simulink model "research_paper_cmrcc"  (R2024b)
settings: Solver=VariableStepAuto  StartTime=0.0  StopTime=0.05  RelTol=1e-3
libraries: spsSeriesRLCBranchLib x9, spsDiodeLib x6, spsCurrentMeasurementLib x5, spsVoltageMeasurementLib x4, spsDCVoltageSourceLib x1, spsGroundLib x1, spsMosfetLib x1, spsMultimeterLib x1, spsMutualInductanceLib x1, eePwmGenerator x1, sps_lib x1
settings Model: Creator=manas  LastModifiedBy=manas

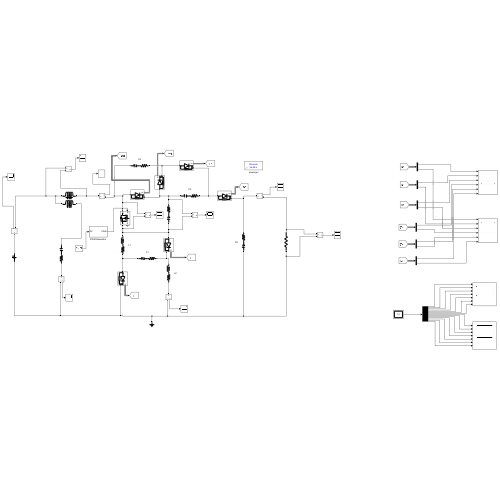
[thumbnail: Simulink's stored preview of the top-level diagram]
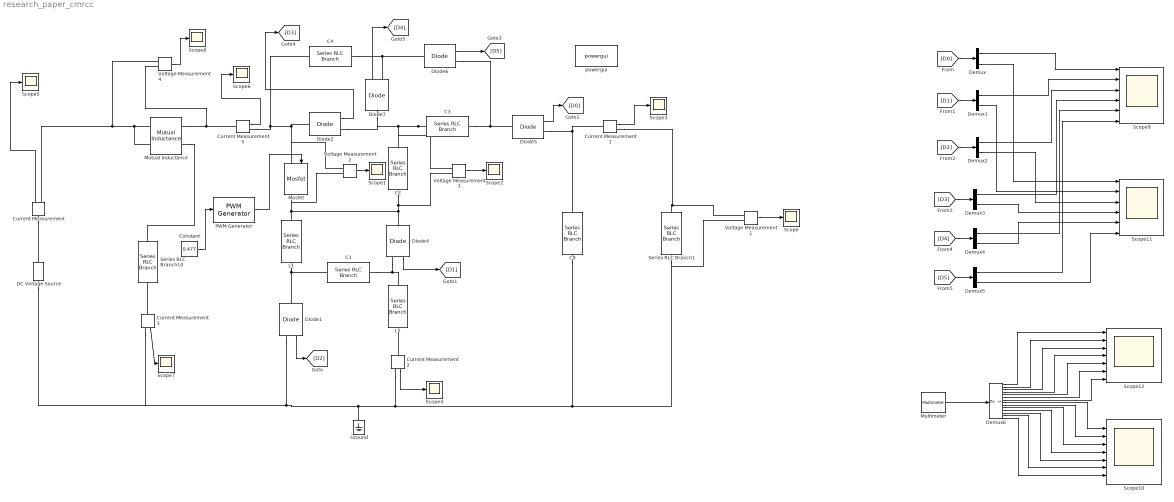
== system research_paper_cmrcc ==
  C0 : spsSeriesRLCBranchLib/Series RLC Branch  LConnTagsString=__new0  RConnTagsString=__new0  BranchType=RC  Resistance=0.05  Inductance=1e-3  SetiL0=off  InitialCurrent=0  Capacitance=100e-6  Setx0=on  InitialVoltage=400  Measurements=Branch voltage and current
  C1 : spsSeriesRLCBranchLib/Series RLC Branch  LConnTagsString=__new0  RConnTagsString=__new0  BranchType=RC  Resistance=0.003  Inductance=1e-3  SetiL0=off  InitialCurrent=0  Capacitance=100e-6  Setx0=on  InitialVoltage=48  Measurements=Branch voltage and current
  C2 : spsSeriesRLCBranchLib/Series RLC Branch  LConnTagsString=__new0  RConnTagsString=__new0  BranchType=RC  Resistance=0.003  Inductance=1e-3  SetiL0=off  InitialCurrent=0  Capacitance=100e-6  Setx0=on  InitialVoltage=176  Measurements=Branch voltage and current
  C3 : spsSeriesRLCBranchLib/Series RLC Branch  LConnTagsString=__new0  RConnTagsString=__new0  BranchType=RC  Resistance=0.003  Inductance=1e-3  SetiL0=off  InitialCurrent=0  Capacitance=100e-6  Setx0=on  InitialVoltage=176  Measurements=Branch voltage and current
  C4 : spsSeriesRLCBranchLib/Series RLC Branch  LConnTagsString=__new0  RConnTagsString=__new0  BranchType=RC  Resistance=0.003  Inductance=1e-3  SetiL0=off  InitialCurrent=0  Capacitance=100e-6  Setx0=on  InitialVoltage=176  Measurements=Branch voltage and current
  Constant : Constant  Value=0.477
  Current Measurement{,1..3,5} (5 alike) : spsCurrentMeasurementLib/Current Measurement  PhasorSimulation=off  OutputType=Complex  PSBequivalent=0
  DC Voltage Source : spsDCVoltageSourceLib/DC Voltage Source  Amplitude=48  Measurements=None
  Demux{,1..5} (6 alike) : Demux  Outputs=2
  Demux6 : Demux  Outputs=14
  Diode1 : spsDiodeLib/Diode  Ron=0.01  Lon=0  Vf=0.85  IC=0  UseSnubber=0  Rs=500  Cs=250e-9  Measurements=on
  Diode{2,5..7} (4 alike) : spsDiodeLib/Diode  Ron=0.01  Lon=0  Vf=0.12  IC=0  UseSnubber=0  Rs=500  Cs=250e-9  Measurements=on
  Diode4 : spsDiodeLib/Diode  Ron=0.01  Lon=0  Vf=0.85  IC=0  UseSnubber=0  Rs=500  Cs=250e-9  Measurements=on
  Ground : spsGroundLib/Ground  LConnTagsString=a
  L1 : spsSeriesRLCBranchLib/Series RLC Branch  LConnTagsString=__new0  RConnTagsString=__new0  BranchType=RL  Resistance=0.12  Inductance=750e-6  SetiL0=on  InitialCurrent=-2.57  Capacitance=1e-6  Setx0=off  InitialVoltage=0  Measurements=Branch voltage and current
  L2 : spsSeriesRLCBranchLib/Series RLC Branch  LConnTagsString=__new0  RConnTagsString=__new0  BranchType=RL  Resistance=0.12  Inductance=750e-6  SetiL0=on  InitialCurrent=-2.57  Capacitance=1e-6  Setx0=off  InitialVoltage=0  Measurements=Branch voltage and current
  Mosfet : spsMosfetLib/Mosfet  Ron=0.016  Lon=0  Rd=0.01  Vfd=0  IC=0  Rs=1e5  Cs=inf  Measurements=on
  Multimeter : spsMultimeterLib/Multimeter  L=14  sel=[1 2 3 4 5 6 7 8 9 10 11 12 13 14]  yselected={}  Gain=[1 1 1 1 1 1 1 1 1 1 1 1 1 1]  OutputType=Complex  PlotAtSimulationStop=off  PhasorSimulation=off
  Mutual Inductance : spsMutualInductanceLib/Mutual Inductance  LConnTagsString=a|b  RConnTagsString=A|B  TypeOfMutual=Two or three windings with equal mutual terms  NumberOfWindings=3  SelfImpedance1=[0.014 1.5e-6]  SelfImpedance2=[0.014 1.5e-6]  ThreeWindings=off  SelfImpedance3=[ 1.1 1.1e-03]  MutualImpedance=[0 1.485e-6]  InductanceMatrix="[1.0 0.9  0.9 ;  0.9 1.0  0.9;  0.9 0.9 1.0 ] * 1e-3"  ResistanceMatrix="[1.0 0.9  0.9 ;  0.9 1.0  0.9;  0.9 0.9 1.0 ]"  Measurements=None
      settings: LibrarySourceBlock=sps_lib/Passives/Mutual Inductance
  PWM Generator : eePwmGenerator/PWM Generator  CarrCount=Up  Tper=25e-6  Tdelay=0  Ts=5e-8
  Scope{,1..8} (9 alike) : Scope
  Scope10 : Scope  NumInputPorts=7
  Scope11 : Scope  NumInputPorts=6
  Scope12 : Scope  NumInputPorts=7
  Scope9 : Scope  NumInputPorts=6
  Series RLC Branch1 : spsSeriesRLCBranchLib/Series RLC Branch  LConnTagsString=__new0  RConnTagsString=__new0  BranchType=R  Resistance=593  Inductance=1e-3  SetiL0=off  InitialCurrent=0  Capacitance=1e-6  Setx0=off  InitialVoltage=0  Measurements=None
  Series RLC Branch10 : spsSeriesRLCBranchLib/Series RLC Branch  LConnTagsString=__new0  RConnTagsString=__new0  BranchType=RC  Resistance=0.0055  Inductance=1.5e-6  SetiL0=off  InitialCurrent=-2.57  Capacitance=1000e-6  Setx0=on  InitialVoltage=-48  Measurements=None
  Voltage Measurement{1..4} (4 alike) : spsVoltageMeasurementLib/Voltage Measurement  PhasorSimulation=off  OutputType=Complex  PSBequivalent=0
  powergui : sps_lib/powergui  Priority=1  SimulationMode=Discrete  SampleTime=5e-8  frequency=60  Iterations=50  frequencyindice=0  Pbase=100e6  ErrMax=1e-4  UnitsV=kV  UnitsW=MW  buscounter=0  FunctionMessages=off  echomessages=off  EnableUseOfTLC=off  CurrentSourceSwitches=off  DisableSnubberDevices=off  DisableRonSwitches=off  DisableVfSwitches=off  DisplayEquations=off  AutomaticDiscreteSolvers=off  SolverType=Tustin/Backward Euler (TBE)  Interpol=off  ExternalGateDelay=off  methode=off  Ts=100  x0status=blocks  SPID=on  SwTol=0  HookPort=off  NonlinearTolerance=1e-4  nMaxIteration=100  ContinueOnMaxIteration=off  RestoreLinks=warning  ResistiveCurrentMeasurement=off  Frange=[0:2:500]  Ylog=off  Xlog=on  ShowGrid=off  save=off  variable=ZData  structure=0  ZoomFFT=off  StartTime=0.0  cycles=1  DisplayStyle=1  fundamental=60  FreqAxis=off  MaxFrequency=1000  frequencyindicesteady=1  RmsSteady=1  display=off
  wires:
  Voltage Measurement2/1 -> Scope1/1
  Constant/1 -> PWM Generator/1
  PWM Generator/1 -> Mosfet/1
  Current Measurement2/1 -> Scope4/1
  Current Measurement/1 -> Scope5/1
  Voltage Measurement1/1 -> Scope/1
  Current Measurement1/1 -> Scope3/1
  Voltage Measurement3/1 -> Scope2/1
  Current Measurement3/1 -> Scope7/1
  Current Measurement5/1 -> Scope6/1
  Voltage Measurement4/1 -> Scope8/1
  Demux6/8 -> Scope10/1
  Demux6/10 -> Scope10/3
  Demux6/1 -> Scope12/1
  Demux6/14 -> Scope10/7
  Demux6/13 -> Scope10/6
  Demux6/4 -> Scope12/4
  Demux6/2 -> Scope12/2
  Demux6/11 -> Scope10/4
  Demux6/6 -> Scope12/6
  Demux6/12 -> Scope10/5
  Demux1/1 -> Scope9/2
  Demux4/1 -> Scope9/5
  Demux5/1 -> Scope9/6
  Demux6/3 -> Scope12/3
  Demux3/2 -> Scope11/4
  Demux1/2 -> Scope11/2
  [D5] -> Demux5/1
  Demux2/2 -> Scope11/3
  [D0] -> Demux/1
  Multimeter/1 -> Demux6/1
  Demux3/1 -> Scope9/4
  Demux2/1 -> Scope9/3
  Demux6/5 -> Scope12/5
  Demux4/2 -> Scope11/5
  [D4] -> Demux4/1
  [D2] -> Demux2/1
  Demux5/2 -> Scope11/6
  Demux6/7 -> Scope12/7
  Demux/2 -> Scope11/1
  Demux6/9 -> Scope10/2
  Demux/1 -> Scope9/1
  [D3] -> Demux3/1
  [D1] -> Demux1/1
  Diode1/1 -> [D2]
  Diode4/1 -> [D1]
  Diode5/1 -> [D0]
  Diode6/1 -> [D5]
  Diode2/1 -> [D3]
  Diode7/1 -> [D4]
  connections:
  C3/LConn1 -- Diode6/RConn1 -- Diode5/LConn1
  Diode1/RConn1 -- Current Measurement2/RConn1 -- C0/RConn1 -- Voltage Measurement1/LConn2 -- Series RLC Branch1/LConn1 -- Ground/LConn1 -- Current Measurement3/RConn1 -- DC Voltage Source/LConn1
  C3/RConn1 -- Diode2/RConn1 -- Diode7/LConn1 -- C2/LConn1 -- Voltage Measurement3/LConn1
  C4/RConn1 -- Voltage Measurement2/LConn1 -- Mosfet/LConn1 -- Diode2/LConn1 -- Current Measurement5/RConn1
  Voltage Measurement1/LConn1 -- Current Measurement1/RConn1 -- Series RLC Branch1/RConn1
  C2/RConn1 -- Diode4/LConn1 -- Voltage Measurement2/LConn2 -- Mosfet/RConn1 -- L1/RConn1 -- Voltage Measurement3/LConn2
  Diode5/RConn1 -- Current Measurement1/LConn1 -- C0/LConn1
  C1/LConn1 -- L2/RConn1 -- Diode4/RConn1
  C1/RConn1 -- Diode1/LConn1 -- L1/LConn1
  Diode7/RConn1 -- C4/LConn1 -- Diode6/LConn1
  Current Measurement2/LConn1 -- L2/LConn1
  Current Measurement/LConn1 -- DC Voltage Source/RConn1
  Mutual Inductance/RConn1 -- Voltage Measurement4/LConn2 -- Current Measurement5/LConn1
  Current Measurement3/LConn1 -- Series RLC Branch10/LConn1
  Current Measurement/RConn1 -- Voltage Measurement4/LConn1 -- Mutual Inductance/LConn2 -- Mutual Inductance/LConn1
  Mutual Inductance/RConn2 -- Series RLC Branch10/RConn1
